simulink model "My_gfm_battery_sil_2_ConvIGBT_zDomain"  (R2025b)
settings: Solver=ode23t  StartTime=0.0  StopTime=10  MaxStep=1e-4  RelTol=1e-3
PreLoadFcn:
  | close all;
  | clear all;
  | clc;
  | 
  | 
  | modelDir = fileparts(get_param(bdroot,'FileName'));
  | 
  | load_system(fullfile(modelDir,'controls_element_lib.slx'));
  | load_system(fullfile(modelDir,'test_sequence_lib.slx'));
  | 
  | Simulink.importExternalCTypes('.\circuitControls_A_autogen.h')
InitFcn:
  | % frequency nominals
  | F_NOM = 60;
  | W_NOM = 2 * pi * F_NOM;
  | 
  | % base values relative to inverter
  | % --------------------------------
  | VLL_INV_NOM = 480;
  | P_INV_NOM = 1e6;
  | Q_INV_NOM = 0.5e6;
  | S_INV_NOM = sqrt(P_INV_NOM^2 + Q_INV_NOM^2);
  | 
  | I_INV_BASE = S_INV_NOM/(sqrt(3)*VLL_INV_NOM);
  | Z_INV_BASE = VLL_INV_NOM^2/S_INV_NOM;
  | L_INV_BASE = Z_INV_BASE / W_NOM;
  | C_INV_BASE = 1 / (Z_INV_BASE * W_NOM);
  | 
  | % nominal ratings for power system model
  | % --------------------------------------
  | INVERTER_COUNT = 100;
  | 
  | VLV_NOM = VLL_INV_NOM;
  | VMV_NOM = 35e3;
  | VHV_NOM = 230e3;
  | S_PLANT = INVERTER_COUNT * S_INV_NOM;
  | 
  | N_GSU = VHV_NOM/VMV_NOM;
  | N_MVT = VMV_NOM/VLV_NOM;
  | 
  | I_LV_BASE = S_PLANT/(sqrt(3)*VLV_NOM);
  | I_MV_BASE = S_PLANT/(sqrt(3)*VMV_NOM);
  | I_HV_BASE = S_PLANT/(sqrt(3)*VHV_NOM);
  | 
  | Z_LV_BASE = VLV_NOM^2/S_PLANT;
  | Z_MV_BASE = VMV_NOM^2/S_PLANT;
  | Z_HV_BASE = VHV_NOM^2/S_PLANT;
  | 
  | L_LV_BASE = Z_LV_BASE / W_NOM;
  | L_MV_BASE = Z_MV_BASE / W_NOM;
  | L_HV_BASE = Z_HV_BASE / W_NOM;
  | C_LV_BASE = 1 / (Z_LV_BASE * W_NOM);
  | C_MV_BASE = 1 / (Z_MV_BASE * W_NOM);
  | C_HV_BASE = 1 / (Z_HV_BASE * W_NOM);
undefined symbols (not defined in the file): D1, D11, Delta, gcbh, j, powergui, SampleTime, sps_rtmsupport, Ts
libraries: simulink x43, spsVoltageMeasurementLib x21, spsThreePhaseSeriesRLCBranchLib x20, spsControlledCurrentSourceLib x20, spsControlledVoltageSourceLib x15, spsThreePhaseVIMeasurementLib x12, spsSeriesRLCBranchLib x11, spsGroundLib x11, test_sequence_lib x10, controls_element_lib x9, spsCurrentMeasurementLib x8, spsThreePhaseTransformerTwoWindingsLib x6
(part 8 of 8)

== system My_gfm_battery_sil_2_ConvIGBT_zDomain/ac Network with MVT (native math)4/Two-Level Converter1/Model3 ==
  note: (Uref)
  g : Inport  SampleTime=Ts
  Block : Inport  Port=2
  Add : Sum  Inputs=+-
  Constant : Constant
  Constant1 : Constant  Value=0
  Constant2 : Constant
  Data Type Conversion2 : DataTypeConversion  OutDataTypeStr=double  SaturateOnIntegerOverflow=off  RndMeth=Floor
  Demux : Demux  Outputs=2
  Fcn2 : Fcn  Expr=(u(1)+1)*0.5
  MATLAB Function : MATLAB Function  TreatAsAtomicUnit=on
  Mux : Mux  Inputs=2
  Mux1 : Mux  Inputs=2
  Power : spsHalfBridgeModel/Power  SystemSampleTime=-1  VariantActivationTime=update diagram  EmptyChoice=off  PassThrough=off  PassThroughVariantControl=(default)  EmptyChoiceVariantControl=(default)  AllowFlexibleInterface=on  Latency=0  AutoFrameSizeCalculation=off
  Product2 : Product
  Product8 : Product
  Saturation : Saturate  UpperLimit=1.0  LowerLimit=-1.0
  Scope : Scope  NumInputPorts=2
      settings: ActiveDisplayYMinimum=-0.125  ActiveDisplayYMaximum=1.125
  Scope1 : Scope  NumInputPorts=2
      settings: ActiveDisplayYMinimum=-0.0256  ActiveDisplayYMaximum=0.96024  DataLoggingVariableName=ScopeData2
  Scope2 : Scope  NumInputPorts=5
      settings: ActiveDisplayYMinimum=-1250  ActiveDisplayYMaximum=1079.00943  DataLoggingVariableName=ScopeData3
  Switch : Switch  Criteria=u2 > Threshold  SaturateOnIntegerOverflow=off  InputSameDT=off
  Transfer Fcn : TransferFcn  Denominator=[1e-6 1]
  Transfer Fcn1 : TransferFcn  Denominator=[1e-6 1]
  Transfer Fcn2 : TransferFcn  Denominator=[1e-6 1]
  Voltage Measurement : spsVoltageMeasurementLib/Voltage Measurement  PhasorSimulation=off  OutputType=Complex  PSBequivalent=0
  + : PMIOPort  Tag=PMCPort  Side=Right
  - : PMIOPort  Tag=PMCPort  Port=2  Side=Right
  Out : PMIOPort  Tag=PMCPort  Port=3  Side=Left
  wires:
  Saturation/1 -> Fcn2/1
  g/1 -> Saturation/1
  Block/1 -> Switch/2, Scope/1
  Data Type Conversion2/1 -> Scope/2, Product2/1, Product8/1
  Product2/1 -> Mux1/1
  Product8/1 -> Mux1/2
  Add/1 -> Scope1/2, Product8/2
  Constant/1 -> Add/1
  Fcn2/1 -> Add/2, Scope1/1, Product2/2
  Switch/1 -> Data Type Conversion2/1
  Power/2 -> Scope2/4, Demux/1
  Demux/2 -> Transfer Fcn2/1
  Demux/1 -> Transfer Fcn/1
  Transfer Fcn/1 -> Mux/1
  Transfer Fcn2/1 -> Mux/2
  Mux/1 -> MATLAB Function/3(I)
  Transfer Fcn1/1 -> MATLAB Function/2(Vdc)
  Power/1 -> Scope2/2, Transfer Fcn1/1
  MATLAB Function/2(Idc) -> Power/2, Scope2/3
  MATLAB Function/1(V) -> Power/1, Scope2/1
  Mux1/1 -> MATLAB Function/1(g)
  Constant1/1 -> Switch/1
  Constant2/1 -> Switch/3
  Voltage Measurement/1 -> Scope2/5
  connections:
  Out/RConn1 -- Power/LConn1 -- Voltage Measurement/LConn1
  -/RConn1 -- Power/RConn2 -- Voltage Measurement/LConn2
  Power/RConn1 -- +/RConn1

== system My_gfm_battery_sil_2_ConvIGBT_zDomain/ac Network with MVT (native math)4/powergui/EquivalentModel1 ==
  Sources : Subsystem
  State-Space : S-Function  FunctionName=sfun_spid_contc  Parameters=S.Mg, [S.nb.x S.nb.u S.nb.y S.nb.s], S.x0, S.MgColNames  SFunctionDeploymentMode=off  EnableBusSupport=off
  Yout : Subsystem
  wires:
  State-Space/1 -> Yout/1(v,i)
  Sources/1(u) -> State-Space/1

== system My_gfm_battery_sil_2_ConvIGBT_zDomain/ac Network with MVT (native math)4/powergui/EquivalentModel2 ==
  Sources : Subsystem
  State-Space : S-Function  FunctionName=sfun_spid_contc  Parameters=S.Mg, [S.nb.x S.nb.u S.nb.y S.nb.s], S.x0, S.MgColNames  SFunctionDeploymentMode=off  EnableBusSupport=off
  Yout : Subsystem
  wires:
  State-Space/1 -> Yout/1(v,i)
  Sources/1(u) -> State-Space/1

== system My_gfm_battery_sil_2_ConvIGBT_zDomain/ac Network with MVT (native math)4/powergui/EquivalentModel3 ==
  Sources : Subsystem
  State-Space : S-Function  FunctionName=sfun_spid_contc  Parameters=S.Mg, [S.nb.x S.nb.u S.nb.y S.nb.s], S.x0, S.MgColNames  SFunctionDeploymentMode=off  EnableBusSupport=off
  Yout : Subsystem
  wires:
  State-Space/1 -> Yout/1(v,i)
  Sources/1(u) -> State-Space/1

== system My_gfm_battery_sil_2_ConvIGBT_zDomain/ac Network with MVT (native math)5/filter_caps/LPF1 ==
  in : Inport
  rst : Inport  Port=2
  Constant : Constant  Value=0
  Constant2 : Constant  Value=Ts
  Delay : Delay  DelayLength=1  InitialCondition=0
  Logical Operator : Logic  Operator=NOT  AllPortsSameDT=off  OutDataTypeStr=boolean
  Product : Product
  Sum : Sum  Inputs=|++
  Switch : Switch  Criteria=u2 ~= 0  SaturateOnIntegerOverflow=off  InputSameDT=off
  out : Outport
  FB : Outport  Port=2
  wires:
  Delay/1 -> Sum/2, FB/1
  Switch/1 -> out/1, Delay/1
  in/1 -> Product/2
  Product/1 -> Sum/1
  Constant2/1 -> Product/1
  Sum/1 -> Switch/1
  Constant/1 -> Switch/3
  rst/1 -> Logical Operator/1
  Logical Operator/1 -> Switch/2

== system My_gfm_battery_sil_2_ConvIGBT_zDomain/ac Network with MVT (native math)5/filter_inductors/LPF1 ==
  in : Inport
  rst : Inport  Port=2
  Constant : Constant  Value=0
  Constant2 : Constant  Value=Ts
  Delay : Delay  DelayLength=1  InitialCondition=0
  Logical Operator : Logic  Operator=NOT  AllPortsSameDT=off  OutDataTypeStr=boolean
  Product : Product
  Sum : Sum  Inputs=|++
  Switch : Switch  Criteria=u2 ~= 0  SaturateOnIntegerOverflow=off  InputSameDT=off
  out : Outport
  FB : Outport  Port=2
  wires:
  Delay/1 -> Sum/2, FB/1
  Switch/1 -> out/1, Delay/1
  in/1 -> Product/2
  Product/1 -> Sum/1
  Constant2/1 -> Product/1
  Sum/1 -> Switch/1
  Constant/1 -> Switch/3
  rst/1 -> Logical Operator/1
  Logical Operator/1 -> Switch/2

== system My_gfm_battery_sil_2_ConvIGBT_zDomain/ac Network with MVT (native math)5/solver_LPF2/LPF1 ==
  in : Inport
  rst : Inport  Port=2
  Constant : Constant  Value=0
  Constant2 : Constant  Value=Ts
  Delay : Delay  DelayLength=1  InitialCondition=0
  Logical Operator : Logic  Operator=NOT  AllPortsSameDT=off  OutDataTypeStr=boolean
  Product : Product
  Sum : Sum  Inputs=|++
  Switch : Switch  Criteria=u2 ~= 0  SaturateOnIntegerOverflow=off  InputSameDT=off
  out : Outport
  FB : Outport  Port=2
  wires:
  Delay/1 -> Sum/2, FB/1
  Switch/1 -> out/1, Delay/1
  in/1 -> Product/2
  Product/1 -> Sum/1
  Constant2/1 -> Product/1
  Sum/1 -> Switch/1
  Constant/1 -> Switch/3
  rst/1 -> Logical Operator/1
  Logical Operator/1 -> Switch/2

== system My_gfm_battery_sil_2_ConvIGBT_zDomain/ac Network with MVT (native math)5/solver_LPF4/LPF1 ==
  in : Inport
  rst : Inport  Port=2
  Constant : Constant  Value=0
  Constant2 : Constant  Value=Ts
  Delay : Delay  DelayLength=1  InitialCondition=0
  Logical Operator : Logic  Operator=NOT  AllPortsSameDT=off  OutDataTypeStr=boolean
  Product : Product
  Sum : Sum  Inputs=|++
  Switch : Switch  Criteria=u2 ~= 0  SaturateOnIntegerOverflow=off  InputSameDT=off
  out : Outport
  FB : Outport  Port=2
  wires:
  Delay/1 -> Sum/2, FB/1
  Switch/1 -> out/1, Delay/1
  in/1 -> Product/2
  Product/1 -> Sum/1
  Constant2/1 -> Product/1
  Sum/1 -> Switch/1
  Constant/1 -> Switch/3
  rst/1 -> Logical Operator/1
  Logical Operator/1 -> Switch/2

== system My_gfm_battery_sil_2_ConvIGBT_zDomain/My Inverter Controller /My_acMonitor_A/Analyzer_V/complex_LPF ==
  note: This was needed because Simulink complains when using transfer functions directly on arrays or complex numbers.
  In1 : Inport
  Complex to Real-Imag : ComplexToRealImag
  Gain2 : Gain  Gain=1/tau
  Gain3 : Gain  Gain=1/tau
  Integrator : Integrator
  Integrator1 : Integrator
  Real-Imag to Complex : RealImagToComplex
  Sum : Sum  Inputs=|+-
  Sum1 : Sum  Inputs=|+-
  Out1 : Outport
  wires:
  Real-Imag to Complex/1 -> Out1/1
  In1/1 -> Complex to Real-Imag/1
  Complex to Real-Imag/1 -> Sum/1
  Integrator/1 -> Real-Imag to Complex/1, Sum/2
  Sum1/1 -> Gain3/1
  Complex to Real-Imag/2 -> Sum1/1
  Gain2/1 -> Integrator/1
  Sum/1 -> Gain2/1
  Integrator1/1 -> Sum1/2, Real-Imag to Complex/2
  Gain3/1 -> Integrator1/1

== system My_gfm_battery_sil_2_ConvIGBT_zDomain/My Inverter Controller /My_acMonitor_A/Analyzer_V1/complex_LPF ==
  note: This was needed because Simulink complains when using transfer functions directly on arrays or complex numbers.
  In1 : Inport
  Complex to Real-Imag : ComplexToRealImag
  Gain2 : Gain  Gain=1/tau
  Gain3 : Gain  Gain=1/tau
  Integrator : Integrator
  Integrator1 : Integrator
  Real-Imag to Complex : RealImagToComplex
  Sum : Sum  Inputs=|+-
  Sum1 : Sum  Inputs=|+-
  Out1 : Outport
  wires:
  Real-Imag to Complex/1 -> Out1/1
  In1/1 -> Complex to Real-Imag/1
  Complex to Real-Imag/1 -> Sum/1
  Integrator/1 -> Real-Imag to Complex/1, Sum/2
  Sum1/1 -> Gain3/1
  Complex to Real-Imag/2 -> Sum1/1
  Gain2/1 -> Integrator/1
  Sum/1 -> Gain2/1
  Integrator1/1 -> Sum1/2, Real-Imag to Complex/2
  Gain3/1 -> Integrator1/1

== system My_gfm_battery_sil_2_ConvIGBT_zDomain/My Inverter Controller /My_acMonitor_A/PLL_3ph/oscillator_3ph ==
  f : Inport
  Cos : Trigonometry  Operator=cos
  Gain : Gain  Gain=2*pi
  Integrator : Integrator
  Real-Imag to Complex : RealImagToComplex
  Sin : Trigonometry
  Sum1 : Sum  Inputs=|++
  phase_shift : Constant  Value=[0 -1/3 -2/3]
  osc[3] : Outport
  wires:
  Sum1/1 -> Gain/1
  phase_shift/1 -> Sum1/2
  Sin/1 -> Real-Imag to Complex/2
  Integrator/1 -> Sum1/1
  Gain/1 -> Sin/1, Cos/1
  Cos/1 -> Real-Imag to Complex/1
  Real-Imag to Complex/1 -> osc[3]/1
  f/1 -> Integrator/1

== system My_gfm_battery_sil_2_ConvIGBT_zDomain/My Inverter Controller /My_circuit_controls_A2/SOGI/Integrator1 ==
  In : Inport
  Ts : Inport  Port=2
  Delay1 : Delay  DelayLength=1
  Delay2 : Delay  DelayLength=1
  Delay3 : Delay  DelayLength=1
  Gain : Gain  Gain=1/12
  Gain1 : Gain  Gain=23
  Gain2 : Gain  Gain=16
  Gain3 : Gain  Gain=5
  Product : Product
  Sum : Sum  Inputs=|+-
  Sum1 : Sum  Inputs=|++
  Sum2 : Sum  Inputs=|++
  Out : Outport  VectorParamsAs1DForOutWhenUnconnected=off
  wires:
  Delay2/1 -> Gain2/1, Delay3/1
  Delay1/1 -> Sum2/2, Gain1/1, Delay2/1
  Delay3/1 -> Gain3/1
  Gain2/1 -> Sum/2
  Gain1/1 -> Sum/1
  Gain3/1 -> Sum1/2
  Sum/1 -> Sum1/1
  Gain/1 -> Sum2/1
  Sum2/1 -> Delay1/1
  Product/1 -> Gain/1
  Sum1/1 -> Out/1
  Ts/1 -> Product/2
  In/1 -> Product/1

== system My_gfm_battery_sil_2_ConvIGBT_zDomain/My Inverter Controller /My_circuit_controls_A2/SOGI/Integrator3 ==
  In : Inport
  Ts : Inport  Port=2
  Delay1 : Delay  DelayLength=1
  Delay2 : Delay  DelayLength=1
  Delay3 : Delay  DelayLength=1
  Gain : Gain  Gain=1/12
  Gain1 : Gain  Gain=23
  Gain2 : Gain  Gain=16
  Gain3 : Gain  Gain=5
  Product : Product
  Sum : Sum  Inputs=|+-
  Sum1 : Sum  Inputs=|++
  Sum2 : Sum  Inputs=|++
  Out : Outport  VectorParamsAs1DForOutWhenUnconnected=off
  wires:
  Delay2/1 -> Gain2/1, Delay3/1
  Delay1/1 -> Sum2/2, Gain1/1, Delay2/1
  Delay3/1 -> Gain3/1
  Gain2/1 -> Sum/2
  Gain1/1 -> Sum/1
  Gain3/1 -> Sum1/2
  Sum/1 -> Sum1/1
  Gain/1 -> Sum2/1
  Sum2/1 -> Delay1/1
  Product/1 -> Gain/1
  Sum1/1 -> Out/1
  Ts/1 -> Product/2
  In/1 -> Product/1

== system My_gfm_battery_sil_2_ConvIGBT_zDomain/My Inverter Controller /My_circuit_controls_A2/Subsystem/LPF4 ==
  note: Forward integrator
  in : Inport
  Constant2 : Constant  Value=Ts
  Constant3 : Constant  Value=OmegaUp
  Constant4 : Constant  Value=OmegaDn
  Constant9 : Constant  Value=1/20000
  Delay : Delay  DelayLength=1  InitialCondition=0
  Gain : Gain  Gain=1/5
  Math Function : Math  Operator=reciprocal  SignedPower=on
  MinMax : MinMax  Function=max  Inputs=2
  MinMax1 : MinMax  Inputs=2
  MinMax2 : MinMax  Inputs=2
  Product : Product
  Product1 : Product
  Product2 : Product
  Saturation : Saturate  UpperLimit=inf  LowerLimit=0
  Saturation1 : Saturate  UpperLimit=0  LowerLimit=-inf
  Sum : Sum  Inputs=|++
  Sum1 : Sum  Inputs=|++
  Sum4 : Sum  Inputs=|+-
  out : Outport
  wires:
  Delay/1 -> Sum4/2, Sum/2
  in/1 -> Sum4/1
  Sum4/1 -> Product2/1, Product1/2
  Sum/1 -> out/1, Delay/1
  Saturation/1 -> Sum1/1
  Saturation1/1 -> Sum1/2
  Sum1/1 -> Product/2
  Product/1 -> Sum/1
  [Ts] -> Product/1
  [OmegaUp] -> Product1/1
  [OmegaDn] -> Product2/2
  Constant2/1 -> MinMax/1
  MinMax/1 -> [Ts]
  Constant9/1 -> MinMax/2
  MinMax1/1 -> [OmegaUp]
  MinMax2/1 -> [OmegaDn]
  [Ts] -> Math Function/1
  Math Function/1 -> Gain/1
  Gain/1 -> MinMax1/2, MinMax2/1
  Constant3/1 -> MinMax1/1
  Constant4/1 -> MinMax2/2
  Product1/1 -> Saturation/1
  Product2/1 -> Saturation1/1

== system My_gfm_battery_sil_2_ConvIGBT_zDomain/My Inverter Controller /My_circuit_controls_A2/virtual damper/Damping HPF ==
  note: Forward integrator
  in : Inport
  Constant2 : Constant  Value=Ts
  Constant3 : Constant  Value=OmegaUp
  Constant4 : Constant  Value=OmegaDn
  Constant9 : Constant  Value=1/20000
  Delay : Delay  DelayLength=1  InitialCondition=0
  Gain : Gain  Gain=1/5
  Math Function : Math  Operator=reciprocal  SignedPower=on
  MinMax : MinMax  Function=max  Inputs=2
  MinMax1 : MinMax  Inputs=2
  MinMax2 : MinMax  Inputs=2
  Product : Product
  Product1 : Product
  Product2 : Product
  Saturation : Saturate  UpperLimit=inf  LowerLimit=0
  Saturation1 : Saturate  UpperLimit=0  LowerLimit=-inf
  Sum : Sum  Inputs=|+-
  Sum1 : Sum  Inputs=|++
  Sum2 : Sum  Inputs=|++
  Sum3 : Sum  Inputs=|+-
  out : Outport  VectorParamsAs1DForOutWhenUnconnected=off
  wires:
  Gain/1 -> MinMax1/2, MinMax2/1
  [Ts] -> Product/1
  [Ts] -> Math Function/1
  Delay/1 -> Sum1/2, Sum/2
  MinMax1/1 -> [OmegaUp]
  Constant9/1 -> MinMax/2
  Sum/1 -> Product2/1, Product1/2
  Math Function/1 -> Gain/1
  Constant4/1 -> MinMax2/2
  Constant2/1 -> MinMax/1
  Saturation/1 -> Sum2/1
  Sum1/1 -> Sum3/2, Delay/1
  Sum2/1 -> Product/2
  MinMax2/1 -> [OmegaDn]
  Product/1 -> Sum1/1
  [OmegaUp] -> Product1/1
  Constant3/1 -> MinMax1/1
  MinMax/1 -> [Ts]
  Product2/1 -> Saturation1/1
  in/1 -> Sum3/1, Sum/1
  Product1/1 -> Saturation/1
  [OmegaDn] -> Product2/2
  Saturation1/1 -> Sum2/2
  Sum3/1 -> out/1

== system My_gfm_battery_sil_2_ConvIGBT_zDomain/My Inverter Controller /My_circuit_controls_A4/SOGI/Integrator1 ==
  In : Inport
  Ts : Inport  Port=2
  Delay1 : Delay  DelayLength=1
  Delay2 : Delay  DelayLength=1
  Delay3 : Delay  DelayLength=1
  Gain : Gain  Gain=1/12
  Gain1 : Gain  Gain=23
  Gain2 : Gain  Gain=16
  Gain3 : Gain  Gain=5
  Product : Product
  Sum : Sum  Inputs=|+-
  Sum1 : Sum  Inputs=|++
  Sum2 : Sum  Inputs=|++
  Out : Outport  VectorParamsAs1DForOutWhenUnconnected=off
  wires:
  Delay2/1 -> Gain2/1, Delay3/1
  Delay1/1 -> Sum2/2, Gain1/1, Delay2/1
  Delay3/1 -> Gain3/1
  Gain2/1 -> Sum/2
  Gain1/1 -> Sum/1
  Gain3/1 -> Sum1/2
  Sum/1 -> Sum1/1
  Gain/1 -> Sum2/1
  Sum2/1 -> Delay1/1
  Product/1 -> Gain/1
  Sum1/1 -> Out/1
  Ts/1 -> Product/2
  In/1 -> Product/1

== system My_gfm_battery_sil_2_ConvIGBT_zDomain/My Inverter Controller /My_circuit_controls_A4/SOGI/Integrator3 ==
  In : Inport
  Ts : Inport  Port=2
  Delay1 : Delay  DelayLength=1
  Delay2 : Delay  DelayLength=1
  Delay3 : Delay  DelayLength=1
  Gain : Gain  Gain=1/12
  Gain1 : Gain  Gain=23
  Gain2 : Gain  Gain=16
  Gain3 : Gain  Gain=5
  Product : Product
  Sum : Sum  Inputs=|+-
  Sum1 : Sum  Inputs=|++
  Sum2 : Sum  Inputs=|++
  Out : Outport  VectorParamsAs1DForOutWhenUnconnected=off
  wires:
  Delay2/1 -> Gain2/1, Delay3/1
  Delay1/1 -> Sum2/2, Gain1/1, Delay2/1
  Delay3/1 -> Gain3/1
  Gain2/1 -> Sum/2
  Gain1/1 -> Sum/1
  Gain3/1 -> Sum1/2
  Sum/1 -> Sum1/1
  Gain/1 -> Sum2/1
  Sum2/1 -> Delay1/1
  Product/1 -> Gain/1
  Sum1/1 -> Out/1
  Ts/1 -> Product/2
  In/1 -> Product/1

== system My_gfm_battery_sil_2_ConvIGBT_zDomain/My Inverter Controller /My_circuit_controls_A4/Subsystem/LPF4 ==
  note: Forward integrator
  in : Inport
  Constant2 : Constant  Value=Ts
  Constant3 : Constant  Value=OmegaUp
  Constant4 : Constant  Value=OmegaDn
  Constant9 : Constant  Value=1/20000
  Delay : Delay  DelayLength=1  InitialCondition=0
  Gain : Gain  Gain=1/5
  Math Function : Math  Operator=reciprocal  SignedPower=on
  MinMax : MinMax  Function=max  Inputs=2
  MinMax1 : MinMax  Inputs=2
  MinMax2 : MinMax  Inputs=2
  Product : Product
  Product1 : Product
  Product2 : Product
  Saturation : Saturate  UpperLimit=inf  LowerLimit=0
  Saturation1 : Saturate  UpperLimit=0  LowerLimit=-inf
  Sum : Sum  Inputs=|++
  Sum1 : Sum  Inputs=|++
  Sum4 : Sum  Inputs=|+-
  out : Outport
  wires:
  Delay/1 -> Sum4/2, Sum/2
  in/1 -> Sum4/1
  Sum4/1 -> Product2/1, Product1/2
  Sum/1 -> out/1, Delay/1
  Saturation/1 -> Sum1/1
  Saturation1/1 -> Sum1/2
  Sum1/1 -> Product/2
  Product/1 -> Sum/1
  [Ts] -> Product/1
  [OmegaUp] -> Product1/1
  [OmegaDn] -> Product2/2
  Constant2/1 -> MinMax/1
  MinMax/1 -> [Ts]
  Constant9/1 -> MinMax/2
  MinMax1/1 -> [OmegaUp]
  MinMax2/1 -> [OmegaDn]
  [Ts] -> Math Function/1
  Math Function/1 -> Gain/1
  Gain/1 -> MinMax1/2, MinMax2/1
  Constant3/1 -> MinMax1/1
  Constant4/1 -> MinMax2/2
  Product1/1 -> Saturation/1
  Product2/1 -> Saturation1/1

== system My_gfm_battery_sil_2_ConvIGBT_zDomain/My Inverter Controller /My_circuit_controls_A4/virtual damper/Damping HPF ==
  note: Forward integrator
  in : Inport
  Constant2 : Constant  Value=Ts
  Constant3 : Constant  Value=OmegaUp
  Constant4 : Constant  Value=OmegaDn
  Constant9 : Constant  Value=1/20000
  Delay : Delay  DelayLength=1  InitialCondition=0
  Gain : Gain  Gain=1/5
  Math Function : Math  Operator=reciprocal  SignedPower=on
  MinMax : MinMax  Function=max  Inputs=2
  MinMax1 : MinMax  Inputs=2
  MinMax2 : MinMax  Inputs=2
  Product : Product
  Product1 : Product
  Product2 : Product
  Saturation : Saturate  UpperLimit=inf  LowerLimit=0
  Saturation1 : Saturate  UpperLimit=0  LowerLimit=-inf
  Sum : Sum  Inputs=|+-
  Sum1 : Sum  Inputs=|++
  Sum2 : Sum  Inputs=|++
  Sum3 : Sum  Inputs=|+-
  out : Outport  VectorParamsAs1DForOutWhenUnconnected=off
  wires:
  Gain/1 -> MinMax1/2, MinMax2/1
  [Ts] -> Product/1
  [Ts] -> Math Function/1
  Delay/1 -> Sum1/2, Sum/2
  MinMax1/1 -> [OmegaUp]
  Constant9/1 -> MinMax/2
  Sum/1 -> Product2/1, Product1/2
  Math Function/1 -> Gain/1
  Constant4/1 -> MinMax2/2
  Constant2/1 -> MinMax/1
  Saturation/1 -> Sum2/1
  Sum1/1 -> Sum3/2, Delay/1
  Sum2/1 -> Product/2
  MinMax2/1 -> [OmegaDn]
  Product/1 -> Sum1/1
  [OmegaUp] -> Product1/1
  Constant3/1 -> MinMax1/1
  MinMax/1 -> [Ts]
  Product2/1 -> Saturation1/1
  in/1 -> Sum3/1, Sum/1
  Product1/1 -> Saturation/1
  [OmegaDn] -> Product2/2
  Saturation1/1 -> Sum2/2
  Sum3/1 -> out/1

== system My_gfm_battery_sil_2_ConvIGBT_zDomain/My Inverter Controller /My_currentLimiting_B/Current_foldback1/LPF  ==
  In : Inport
  1/0.01 : Gain  Gain=1/0.01
  Integrator : Integrator
  Sum3 : Sum  Inputs=|+-
  Out : Outport
  wires:
  Integrator/1 -> Out/1, Sum3/2
  Sum3/1 -> 1/0.01/1
  In/1 -> Sum3/1
  1/0.01/1 -> Integrator/1

== system My_gfm_battery_sil_2_ConvIGBT_zDomain/My Inverter Controller /My_machineModel_A/AVR/ Saturation ==
  In : Inport
  Complex to Real-Imag : ComplexToRealImag
  Real-Imag to Complex3 : RealImagToComplex
  Saturation3 : Saturate  UpperLimit=0.1*VllRated  LowerLimit=-0.1*VllRated
  Saturation4 : Saturate  UpperLimit=0.1*VllRated  LowerLimit=-0.1*VllRated
  Out : Outport  VectorParamsAs1DForOutWhenUnconnected=off
  wires:
  Complex to Real-Imag/1 -> Saturation3/1
  Saturation4/1 -> Real-Imag to Complex3/2
  Complex to Real-Imag/2 -> Saturation4/1
  Saturation3/1 -> Real-Imag to Complex3/1
  In/1 -> Complex to Real-Imag/1
  Real-Imag to Complex3/1 -> Out/1

== system My_gfm_battery_sil_2_ConvIGBT_zDomain/My Inverter Controller /My_machineModel_A/AVR/LPF ==
  In : Inport
  1/tauMeas : Gain  Gain=1/tauMeas
  Integrator : Integrator
  Sum3 : Sum  Inputs=|+-
  Out : Outport
  wires:
  Integrator/1 -> Out/1, Sum3/2
  Sum3/1 -> 1/tauMeas/1
  In/1 -> Sum3/1
  1/tauMeas/1 -> Integrator/1

== system My_gfm_battery_sil_2_ConvIGBT_zDomain/My Inverter Controller /My_machineModel_A/AVR/LPF  ==
  In : Inport
  1/tauMeas : Gain  Gain=1/tauMeas
  Integrator : Integrator
  Sum3 : Sum  Inputs=|+-
  Out : Outport
  wires:
  Integrator/1 -> Out/1, Sum3/2
  Sum3/1 -> 1/tauMeas/1
  In/1 -> Sum3/1
  1/tauMeas/1 -> Integrator/1

== system My_gfm_battery_sil_2_ConvIGBT_zDomain/My Inverter Controller /My_machineModel_A/AVR/LPF   ==
  In : Inport
  1/tauMeas : Gain  Gain=1/tauMeas
  Integrator : Integrator
  Sum3 : Sum  Inputs=|+-
  Out : Outport
  wires:
  Integrator/1 -> Out/1, Sum3/2
  Sum3/1 -> 1/tauMeas/1
  In/1 -> Sum3/1
  1/tauMeas/1 -> Integrator/1

== system My_gfm_battery_sil_2_ConvIGBT_zDomain/My Inverter Controller /My_machineModel_A/AVR/assymmetric filter ==
  note: The saturation block is configured to cause a rapid rise, but much slow drop in output.
  in : Inport
  Gain1 : Gain  Gain=1/tauBkSt
  Integrator : Integrator
  Saturation1 : Saturate  UpperLimit=VllRated  LowerLimit=-0.02 * VllRated
  Sum3 : Sum  Inputs=|+-
  out : Outport
  wires:
  Saturation1/1 -> Integrator/1
  Gain1/1 -> Saturation1/1
  in/1 -> Sum3/1
  Sum3/1 -> Gain1/1
  Integrator/1 -> Sum3/2, out/1

== system My_gfm_battery_sil_2_ConvIGBT_zDomain/My Inverter Controller /My_machineModel_A/AVR/current analyzer ==
  osc[3] : Inport
  iac : Inport  Port=2
  Complex to Real-Imag : ComplexToRealImag
  Conj : Math  Operator=conj  SignedPower=on
  Product1 : Product
  Product2 : Product
  Sum of Elements1 : Sum  Inputs=+
  Sum of Elements2 : Sum  Inputs=+
  Transfer Fcn : TransferFcn  Denominator=[0.02 1]
  Transfer Fcn1 : TransferFcn  Denominator=[0.02 1]
  over_sqrt(3) : Gain  Gain=1/sqrt(3)
  over_sqrt(3)1 : Gain  Gain=1/sqrt(3)
  sqrt(2) : Gain  Gain=sqrt(2)
  Id : Outport
  Iq : Outport  Port=2
  wires:
  Transfer Fcn/1 -> Iq/1
  osc[3]/1 -> Conj/1
  Transfer Fcn1/1 -> Id/1
  over_sqrt(3)1/1 -> Transfer Fcn1/1
  over_sqrt(3)/1 -> Transfer Fcn/1
  Complex to Real-Imag/1 -> Product2/1
  Complex to Real-Imag/2 -> Product1/1
  Sum of Elements2/1 -> over_sqrt(3)1/1
  iac/1 -> Product2/2, Product1/2
  Product1/1 -> Sum of Elements1/1
  Sum of Elements1/1 -> over_sqrt(3)/1
  sqrt(2)/1 -> Complex to Real-Imag/1
  Conj/1 -> sqrt(2)/1
  Product2/1 -> Sum of Elements2/1

== system My_gfm_battery_sil_2_ConvIGBT_zDomain/My Inverter Controller /My_machineModel_A/Exciter/LPF ==
  In : Inport
  Integrator : Integrator
  Sum3 : Sum  Inputs=|+-
  wExciter : Gain  Gain=wExciter
  Out : Outport
  wires:
  Integrator/1 -> Out/1, Sum3/2
  Sum3/1 -> wExciter/1
  In/1 -> Sum3/1
  wExciter/1 -> Integrator/1

== system My_gfm_battery_sil_2_ConvIGBT_zDomain/My Inverter Controller /My_machineModel_A/Exciter/modulator ==
  cmd : Inport
  osc : Inport  Port=2
  Complex to Real-Imag : ComplexToRealImag
  Complex to Real-Imag1 : ComplexToRealImag
  Gain : Gain  Gain=sqrt(2)
  Product1 : Product
  Product2 : Product
  Sum1 : Sum  Inputs=|+-
  ref : Outport
  wires:
  osc/1 -> Gain/1
  Complex to Real-Imag/1 -> Product2/2
  Product2/1 -> Sum1/1
  Sum1/1 -> ref/1  "i"
  Gain/1 -> Complex to Real-Imag/1
  Complex to Real-Imag/2 -> Product1/2
  Product1/1 -> Sum1/2
  cmd/1 -> Complex to Real-Imag1/1
  Complex to Real-Imag1/1 -> Product2/1
  Complex to Real-Imag1/2 -> Product1/1

== system My_gfm_battery_sil_2_ConvIGBT_zDomain/My Inverter Controller /My_machineModel_A/governer/LPF(DamperDecoupler) limited  ==
  In : Inport
  Constant : Constant  Value=1/tau_damp
  Constant1 : Constant  Value=wGoverner
  Integrator : Integrator  LimitOutput=on  UpperSaturationLimit=1.2*SRated  LowerSaturationLimit=-1.2*SRated
  MinMax : MinMax  Inputs=2
  Product : Product
  Sum3 : Sum  Inputs=|+-
  Out : Outport
  wires:
  Integrator/1 -> Out/1, Sum3/2
  Sum3/1 -> Product/2
  In/1 -> Sum3/1
  Product/1 -> Integrator/1
  MinMax/1 -> Product/1
  Constant/1 -> MinMax/1
  Constant1/1 -> MinMax/2

== system My_gfm_battery_sil_2_ConvIGBT_zDomain/My Inverter Controller /My_machineModel_A/governer/synchronizer ==
  note: Big Range?
  note: prevent it from acting during typical faults
  note: Prevent loss of sync at low voltage events, using asym filter to traget long extended low voltage events
  note: Keeps the machine spining in synchronize while machine is disabled, disabling the machine means
  note: Why?
  Vq : Inport
  Vt : Inport  Port=2
  machine_enabled : Inport  Port=3
  Constant : Constant
  Gain : Gain  Gain=SRated
  Gain2 : Gain  Gain=1/VllRated
  "HPF " : Subsystem
  Product1 : Product
  Saturation : Saturate  UpperLimit=1  LowerLimit=0
  Sum : Sum  Inputs=|++
  Sum2 : Sum  Inputs=|+-
  Switch : Switch  Criteria=u2 > Threshold  SaturateOnIntegerOverflow=off  InputSameDT=off
  assymmetric filter1 : Subsystem
  gain : Gain  Gain=wSync
  kFastSync : Gain  Gain=kpFastSync
  kSync : Gain  Gain=kpSync
  pSyncLimit : Saturate  UpperLimit=3  LowerLimit=-3
  syncFadeGain : Gain  Gain=kpSyncFade
  syncFadeThreshold : Constant  Value=SyncFadeThres
  to_pu : Gain  Gain=1 / VllRated
  p_sync_pu : Outport
  wires:
  to_pu/1 -> Sum2/2
  Vt/1 -> assymmetric filter1/1(in)
  assymmetric filter1/1(out) -> to_pu/1
  pSyncLimit/1 -> Gain/1
  kSync/1 -> Sum/1
  Sum/1 -> pSyncLimit/1
  Product1/1 -> p_sync_pu/1
  Constant/1 -> Switch/3
  Sum2/1 -> syncFadeGain/1
  machine_enabled/1 -> Switch/2
  syncFadeGain/1 -> Saturation/1
  Saturation/1 -> Switch/1
  syncFadeThreshold/1 -> Sum2/1
  Switch/1 -> Product1/2
  Gain2/1 -> kFastSync/1, kSync/1
  Vq/1 -> Gain2/1
  Gain/1 -> Product1/1  "p_sync"
  kFastSync/1 -> "HPF "/1(in)
  "HPF "/1(out) -> gain/1
  gain/1 -> Sum/2

== system My_gfm_battery_sil_2_ConvIGBT_zDomain/My Inverter Controller /My_machineModel_A/rotor model/HPF (wDamperDecoupler) 1 ==
  in : Inport
  1/tau_damp : Gain  Gain=1/tau_damp
  Integrator : Integrator
  Sum : Sum  Inputs=|+-
  out : Outport
  wires:
  Sum/1 -> out/1, 1/tau_damp/1
  in/1 -> Sum/1
  Integrator/1 -> Sum/2
  1/tau_damp/1 -> Integrator/1

== system My_gfm_battery_sil_2_ConvIGBT_zDomain/My Inverter Controller /My_machineModel_A/rotor model/oscillator_3ph ==
  f : Inport
  Cos : Trigonometry  Operator=cos
  Gain : Gain  Gain=2*pi
  Integrator : Integrator
  Real-Imag to Complex : RealImagToComplex
  Sin : Trigonometry
  Sum1 : Sum  Inputs=|++
  phase_shift : Constant  Value=[0 -1/3 -2/3]
  osc[3] : Outport
  wires:
  f/1 -> Integrator/1
  Real-Imag to Complex/1 -> osc[3]/1
  Cos/1 -> Real-Imag to Complex/1
  Gain/1 -> Cos/1, Sin/1
  Integrator/1 -> Sum1/1
  Sin/1 -> Real-Imag to Complex/2
  phase_shift/1 -> Sum1/2
  Sum1/1 -> Gain/1

== system My_gfm_battery_sil_2_ConvIGBT_zDomain/My Inverter Controller /My_machineModel_A/voltage analyzer/LPF ==
  In : Inport
  1/tauMeas : Gain  Gain=1/tauMeas
  Integrator : Integrator
  Sum3 : Sum  Inputs=|+-
  Out : Outport
  wires:
  Integrator/1 -> Out/1, Sum3/2
  Sum3/1 -> 1/tauMeas/1
  In/1 -> Sum3/1
  1/tauMeas/1 -> Integrator/1

== system My_gfm_battery_sil_2_ConvIGBT_zDomain/My Inverter Controller /My_machineModel_A/voltage analyzer/LPF  ==
  In : Inport
  1/tauMeas : Gain  Gain=1/tauMeas
  Integrator : Integrator
  Sum3 : Sum  Inputs=|+-
  Out : Outport
  wires:
  Integrator/1 -> Out/1, Sum3/2
  Sum3/1 -> 1/tauMeas/1
  In/1 -> Sum3/1
  1/tauMeas/1 -> Integrator/1

== system My_gfm_battery_sil_2_ConvIGBT_zDomain/My Inverter Controller /My_machineModel_A1/excitation/LPF ==
  In : Inport
  Integrator : Integrator
  Sum3 : Sum  Inputs=|+-
  wExciter : Gain  Gain=wExciter
  Out : Outport
  wires:
  Integrator/1 -> Out/1, Sum3/2
  Sum3/1 -> wExciter/1
  In/1 -> Sum3/1
  wExciter/1 -> Integrator/1

== system My_gfm_battery_sil_2_ConvIGBT_zDomain/My Inverter Controller /My_machineModel_A1/excitation/assymmetric filter1 ==
  note: The saturation block is configured to cause a rapid rise, but much slow drop in output.
  in : Inport
  Gain1 : Gain  Gain=2
  Integrator : Integrator
  Saturation1 : Saturate  UpperLimit=VllRated  LowerLimit=-0.02 * VllRated
  Sum3 : Sum  Inputs=|+-
  out : Outport
  wires:
  Saturation1/1 -> Integrator/1
  Gain1/1 -> Saturation1/1
  in/1 -> Sum3/1
  Sum3/1 -> Gain1/1
  Integrator/1 -> Sum3/2, out/1

== system My_gfm_battery_sil_2_ConvIGBT_zDomain/My Inverter Controller /My_machineModel_A1/excitation/modulator ==
  cmd : Inport
  osc : Inport  Port=2
  Complex to Real-Imag : ComplexToRealImag
  Complex to Real-Imag1 : ComplexToRealImag
  Gain : Gain  Gain=sqrt(2)
  Product1 : Product
  Product2 : Product
  Sum1 : Sum  Inputs=|+-
  ref : Outport
  wires:
  osc/1 -> Gain/1
  Complex to Real-Imag/1 -> Product2/2
  Product2/1 -> Sum1/1
  Sum1/1 -> ref/1  "i"
  Gain/1 -> Complex to Real-Imag/1
  Complex to Real-Imag/2 -> Product1/2
  Product1/1 -> Sum1/2
  cmd/1 -> Complex to Real-Imag1/1
  Complex to Real-Imag1/1 -> Product2/1
  Complex to Real-Imag1/2 -> Product1/1

== system My_gfm_battery_sil_2_ConvIGBT_zDomain/My Inverter Controller /My_machineModel_A1/governer/LPF(DamperDecoupler) limited  ==
  In : Inport
  1/tau_damp : Gain  Gain=1/0.3
  Integrator : Integrator  LimitOutput=on  UpperSaturationLimit=1.2*SRated  LowerSaturationLimit=-1.2*SRated
  Sum3 : Sum  Inputs=|+-
  Out : Outport
  wires:
  Integrator/1 -> Out/1, Sum3/2
  Sum3/1 -> 1/tau_damp/1
  In/1 -> Sum3/1
  1/tau_damp/1 -> Integrator/1

== system My_gfm_battery_sil_2_ConvIGBT_zDomain/My Inverter Controller /My_machineModel_A1/governer/synchronizer ==
  note: Why?
  note: Big Range?
  note: prevent it from acting during typical faults
  note: Prevent loss of sync at low voltage events, using asym filter to traget long extended low voltage events
  note: Keeps the machine spining in synchronize while machine is disabled, disabling the machine means
  note: Why?
  Vq : Inport
  Vt : Inport  Port=2
  machine_enabled : Inport  Port=3
  Constant : Constant
  Gain : Gain  Gain=SRated
  Gain2 : Gain  Gain=1/VllRated
  HPF : Subsystem
  Product1 : Product
  Saturation : Saturate  UpperLimit=1  LowerLimit=0
  Sum : Sum  Inputs=|++
  Sum2 : Sum  Inputs=|+-
  Switch : Switch  Criteria=u2 > Threshold  SaturateOnIntegerOverflow=off  InputSameDT=off
  Transfer Fcn : TransferFcn  Commented=on  Numerator=[(2 * pi * 50) 0]  Denominator=[1, (2*pi*50)]
  assymmetric filter1 : Subsystem
  gain : Gain  Gain=2*pi*50
  kFastSync : Gain
  kSync : Gain  Gain=20
  pSyncLimit : Saturate  UpperLimit=3  LowerLimit=-3
  syncFadeGain : Gain  Gain=4
  syncFadeThreshold : Constant  Value=0.2
  to_pu : Gain  Gain=1 / VllRated
  p_sync_pu : Outport
  wires:
  to_pu/1 -> Sum2/2
  Vt/1 -> assymmetric filter1/1(in)
  assymmetric filter1/1(out) -> to_pu/1
  pSyncLimit/1 -> Gain/1
  kSync/1 -> Sum/1
  Sum/1 -> pSyncLimit/1
  Product1/1 -> p_sync_pu/1
  Constant/1 -> Switch/3
  Sum2/1 -> syncFadeGain/1
  machine_enabled/1 -> Switch/2
  syncFadeGain/1 -> Saturation/1
  Saturation/1 -> Switch/1
  syncFadeThreshold/1 -> Sum2/1
  Switch/1 -> Product1/2
  Gain2/1 -> kFastSync/1, kSync/1
  Vq/1 -> Gain2/1
  Gain/1 -> Product1/1  "p_sync"
  kFastSync/1 -> HPF/1(in)
  HPF/1(out) -> gain/1
  gain/1 -> Sum/2

== system My_gfm_battery_sil_2_ConvIGBT_zDomain/My Inverter Controller /My_machineModel_A1/governer1/LPF(DamperDecoupler) - limited ==
  In1 : Inport
  Integrator : Integrator  LimitOutput=on  UpperSaturationLimit=1.2*SRated  LowerSaturationLimit=-1.2*SRated
  Sum3 : Sum  Inputs=|+-
  wDamperDecoupler : Gain  Gain=1/0.3
  Out1 : Outport
  wires:
  Integrator/1 -> Out1/1, Sum3/2
  Sum3/1 -> wDamperDecoupler/1
  wDamperDecoupler/1 -> Integrator/1
  In1/1 -> Sum3/1

== system My_gfm_battery_sil_2_ConvIGBT_zDomain/My Inverter Controller /My_machineModel_A1/governer1/LPF(DamperDecoupler) limited 1 ==
  In : Inport
  1/tau_damp : Gain  Gain=1/0.3
  Integrator : Integrator  LimitOutput=on  UpperSaturationLimit=1.2*SRated  LowerSaturationLimit=-1.2*SRated
  Sum3 : Sum  Inputs=|+-
  Out : Outport
  wires:
  Integrator/1 -> Out/1, Sum3/2
  Sum3/1 -> 1/tau_damp/1
  In/1 -> Sum3/1
  1/tau_damp/1 -> Integrator/1

== system My_gfm_battery_sil_2_ConvIGBT_zDomain/My Inverter Controller /My_machineModel_A1/governer1/synchronizer ==
  note: Why?
  note: Big Range?
  note: prevent it from acting during typical faults
  note: Prevent loss of sync at low voltage events, using asym filter to traget long extended low voltage events
  note: Keeps the machine spining in synchronize while machine is disabled, disabling the machine means
  note: Why?
  note: Should be sqrt(Vd^2 + Vq^2) ?
  Vq : Inport
  Vd : Inport  Port=2
  machine_enabled : Inport  Port=3
  Constant : Constant
  Gain : Gain  Gain=SRated
  Gain2 : Gain  Gain=1/VllRated
  HPF : Subsystem
  Product1 : Product
  Saturation : Saturate  UpperLimit=1  LowerLimit=0
  Sum : Sum  Inputs=|++
  Sum2 : Sum  Inputs=|+-
  Switch : Switch  Criteria=u2 > Threshold  SaturateOnIntegerOverflow=off  InputSameDT=off
  Transfer Fcn : TransferFcn  Commented=on  Numerator=[(2 * pi * 50) 0]  Denominator=[1, (2*pi*50)]
  assymmetric filter1 : Subsystem
  gain : Gain  Gain=2*pi*50
  kFastSync : Gain
  kSync : Gain  Gain=20
  pSyncLimit : Saturate  UpperLimit=3  LowerLimit=-3
  syncFadeGain : Gain  Gain=4
  syncFadeThreshold : Constant  Value=0.2
  to_pu : Gain  Gain=1 / VllRated
  p_sync_pu : Outport
  wires:
  to_pu/1 -> Sum2/2
  Vd/1 -> assymmetric filter1/1(in)
  assymmetric filter1/1(out) -> to_pu/1
  pSyncLimit/1 -> Gain/1
  kSync/1 -> Sum/1
  Sum/1 -> pSyncLimit/1
  Product1/1 -> p_sync_pu/1
  Constant/1 -> Switch/3
  Sum2/1 -> syncFadeGain/1
  machine_enabled/1 -> Switch/2
  syncFadeGain/1 -> Saturation/1
  Saturation/1 -> Switch/1
  syncFadeThreshold/1 -> Sum2/1
  Switch/1 -> Product1/2
  Gain2/1 -> kFastSync/1, kSync/1
  Vq/1 -> Gain2/1
  Gain/1 -> Product1/1  "p_sync"
  kFastSync/1 -> HPF/1(in)
  HPF/1(out) -> gain/1
  gain/1 -> Sum/2

== system My_gfm_battery_sil_2_ConvIGBT_zDomain/My Inverter Controller /My_machineModel_A1/rotor model/HPF (wDamperDecoupler) 1 ==
  in : Inport
  1/tau_damp : Gain  Gain=1/0.3
  Integrator : Integrator
  Sum : Sum  Inputs=|+-
  out : Outport
  wires:
  Sum/1 -> out/1, 1/tau_damp/1
  in/1 -> Sum/1
  Integrator/1 -> Sum/2
  1/tau_damp/1 -> Integrator/1

== system My_gfm_battery_sil_2_ConvIGBT_zDomain/My Inverter Controller /My_machineModel_A1/rotor model/oscillator_3ph ==
  f : Inport
  Cos : Trigonometry  Operator=cos
  Gain : Gain  Gain=2*pi
  Integrator : Integrator
  Real-Imag to Complex : RealImagToComplex
  Sin : Trigonometry
  Sum1 : Sum  Inputs=|++
  phase_shift : Constant  Value=[0 -1/3 -2/3]
  osc[3] : Outport
  wires:
  f/1 -> Integrator/1
  Real-Imag to Complex/1 -> osc[3]/1
  Cos/1 -> Real-Imag to Complex/1
  Gain/1 -> Cos/1, Sin/1
  Integrator/1 -> Sum1/1
  Sin/1 -> Real-Imag to Complex/2
  phase_shift/1 -> Sum1/2
  Sum1/1 -> Gain/1

== system My_gfm_battery_sil_2_ConvIGBT_zDomain/Plant controller (simplified example)/Meter/PLL-analog/oscillator_3ph ==
  f : Inport
  Cos : Trigonometry  Operator=cos
  Gain : Gain  Gain=2*pi
  Integrator : Integrator
  Real-Imag to Complex : RealImagToComplex
  Sin : Trigonometry
  Sum1 : Sum  Inputs=|++
  phase_shift : Constant  Value=[0 -1/3 -2/3]
  osc[3] : Outport
  wires:
  Sum1/1 -> Gain/1
  phase_shift/1 -> Sum1/2
  Sin/1 -> Real-Imag to Complex/2
  Integrator/1 -> Sum1/1
  Gain/1 -> Sin/1, Cos/1
  Cos/1 -> Real-Imag to Complex/1
  Real-Imag to Complex/1 -> osc[3]/1
  f/1 -> Integrator/1

== system My_gfm_battery_sil_2_ConvIGBT_zDomain/ac Network with MVT (native math)4/powergui/EquivalentModel1/Sources ==
  Mux : Mux  Inputs=[1 1 1 1 1 1]
  u : Outport  VectorParamsAs1DForOutWhenUnconnected=off
  wires:
  Mux/1 -> u/1
  [T110_10072_18540693045835] -> Mux/1
  [T110_10073_18546958997832] -> Mux/2
  [T110_10074_18553562230555] -> Mux/3
  [T104_9471_15257157992367] -> Mux/4
  [T104_9472_15263231413055] -> Mux/5
  [T105_9521_15201317903447] -> Mux/6

== system My_gfm_battery_sil_2_ConvIGBT_zDomain/ac Network with MVT (native math)4/powergui/EquivalentModel1/Yout ==
  v,i : Inport
  Demux : Demux  Outputs=[1 1 1 1 1 1 1 1 1 1 1 1 1 1 1 1 1]
  tag scope: T101_8788_13506312305887=global, T101_8789_13512331616667=global, T101_8790_13518638934576=global, T101_8800_13617096052105=global, T101_8801_13623081547123=global, T101_8802_13629355049269=global, T102_8863_13653826365305=global, T102_8864_13659950384888=global, T102_8865_13666365769374=global, T102_8875_13766394121088=global, T102_8876_13772484261417=global, T102_8877_13778865766648=global, T114_10480_19873251167167=global, T114_10482_19885120530449=global, T127_11890_28685161815829=global, T128_11939_28594174590354=global, T128_11940_28594194970608=global
  wires:
  v,i/1 -> Demux/1
  Demux/1 -> [T102_8875_13766394121088]
  Demux/2 -> [T102_8876_13772484261417]
  Demux/3 -> [T102_8877_13778865766648]
  Demux/4 -> [T101_8800_13617096052105]
  Demux/5 -> [T101_8801_13623081547123]
  Demux/6 -> [T101_8802_13629355049269]
  Demux/7 -> [T114_10480_19873251167167]
  Demux/8 -> [T114_10482_19885120530449]
  Demux/9 -> [T102_8863_13653826365305]
  Demux/10 -> [T102_8864_13659950384888]
  Demux/11 -> [T102_8865_13666365769374]
  Demux/12 -> [T101_8788_13506312305887]
  Demux/13 -> [T101_8789_13512331616667]
  Demux/14 -> [T101_8790_13518638934576]
  Demux/15 -> [T127_11890_28685161815829]
  Demux/16 -> [T128_11939_28594174590354]
  Demux/17 -> [T128_11940_28594194970608]

== system My_gfm_battery_sil_2_ConvIGBT_zDomain/ac Network with MVT (native math)4/powergui/EquivalentModel2/Sources ==
  Mux : Mux  Inputs=[1 1 1 1 1 1]
  u : Outport  VectorParamsAs1DForOutWhenUnconnected=off
  wires:
  Mux/1 -> u/1
  [T127_11776_26356052463873] -> Mux/1
  [T128_11825_26229814574488] -> Mux/2
  [T85_7683_9614987755625] -> Mux/3
  [T85_7684_9619946320720] -> Mux/4
  [T85_7685_9615963782852] -> Mux/5
  [T85_7686_9620916550042] -> Mux/6

== system My_gfm_battery_sil_2_ConvIGBT_zDomain/ac Network with MVT (native math)4/powergui/EquivalentModel2/Yout ==
  v,i : Inport
  Demux : Demux  Outputs=[1 1 1 1 1 1 1 1 1 1 1 1 1 1 1 1 1 1]
  tag scope: T101_8844_13845888351347=global, T101_8845_13851766681921=global, T101_8846_13857933019624=global, T101_8856_13955016807584=global, T101_8857_13960861322396=global, T101_8858_13966993844337=global, T102_8884_13951931031537=global, T102_8885_13957994439534=global, T102_8886_13964349212434=global, T102_8896_14063786961671=global, T102_8897_14069816490414=global, T102_8898_14076137384058=global, T127_11925_28478252064881=global, T128_11974_28388591653140=global, T128_11975_28388555561297=global, T94_8644_13498791624137=global, T94_8646_13507986467916=global, T95_8695_13502152486009=global
  wires:
  v,i/1 -> Demux/1
  Demux/1 -> [T102_8896_14063786961671]
  Demux/2 -> [T102_8897_14069816490414]
  Demux/3 -> [T102_8898_14076137384058]
  Demux/4 -> [T101_8856_13955016807584]
  Demux/5 -> [T101_8857_13960861322396]
  Demux/6 -> [T101_8858_13966993844337]
  Demux/7 -> [T94_8644_13498791624137]
  Demux/8 -> [T94_8646_13507986467916]
  Demux/9 -> [T95_8695_13502152486009]
  Demux/10 -> [T102_8884_13951931031537]
  Demux/11 -> [T102_8885_13957994439534]
  Demux/12 -> [T102_8886_13964349212434]
  Demux/13 -> [T101_8844_13845888351347]
  Demux/14 -> [T101_8845_13851766681921]
  Demux/15 -> [T101_8846_13857933019624]
  Demux/16 -> [T127_11925_28478252064881]
  Demux/17 -> [T128_11974_28388591653140]
  Demux/18 -> [T128_11975_28388555561297]

== system My_gfm_battery_sil_2_ConvIGBT_zDomain/ac Network with MVT (native math)4/powergui/EquivalentModel3/Sources ==
  Mux : Mux  Inputs=[1 1]
  u : Outport  VectorParamsAs1DForOutWhenUnconnected=off
  wires:
  Mux/1 -> u/1
  [T103_9651_17767016193933] -> Mux/1
  [T108_9898_18128775488598] -> Mux/2

== system My_gfm_battery_sil_2_ConvIGBT_zDomain/ac Network with MVT (native math)4/powergui/EquivalentModel3/Yout ==
  v,i : Inport
  Demux : Demux  Outputs=[1 1]
  tag scope: T112_10295_19938657508366=global, T99_9354_17225524064677=global
  wires:
  v,i/1 -> Demux/1
  Demux/1 -> [T112_10295_19938657508366]
  Demux/2 -> [T99_9354_17225524064677]

== system My_gfm_battery_sil_2_ConvIGBT_zDomain/My Inverter Controller /My_machineModel_A/governer/synchronizer/HPF  ==
  in : Inport
  Integrator : Integrator
  Sum : Sum  Inputs=|+-
  wSync : Gain  Gain=wSync
  out : Outport
  wires:
  Sum/1 -> out/1, wSync/1
  in/1 -> Sum/1
  Integrator/1 -> Sum/2
  wSync/1 -> Integrator/1

== system My_gfm_battery_sil_2_ConvIGBT_zDomain/My Inverter Controller /My_machineModel_A/governer/synchronizer/assymmetric filter1 ==
  note: The saturation block is configured to cause a rapid rise, but much slow drop in output.
  in : Inport
  Gain1 : Gain  Gain=1/tauBkSt
  Integrator : Integrator
  Saturation1 : Saturate  UpperLimit=VllRated  LowerLimit=-0.02 * VllRated
  Sum3 : Sum  Inputs=|+-
  out : Outport
  wires:
  Integrator/1 -> out/1, Sum3/2
  Sum3/1 -> Gain1/1
  in/1 -> Sum3/1
  Gain1/1 -> Saturation1/1
  Saturation1/1 -> Integrator/1

== system My_gfm_battery_sil_2_ConvIGBT_zDomain/My Inverter Controller /My_machineModel_A1/governer/synchronizer/HPF ==
  in : Inport
  1/tau : Gain  Gain=2*pi*50
  Integrator : Integrator
  Sum : Sum  Inputs=|+-
  out : Outport
  wires:
  Sum/1 -> out/1, 1/tau/1
  in/1 -> Sum/1
  Integrator/1 -> Sum/2
  1/tau/1 -> Integrator/1

== system My_gfm_battery_sil_2_ConvIGBT_zDomain/My Inverter Controller /My_machineModel_A1/governer/synchronizer/assymmetric filter1 ==
  note: The saturation block is configured to cause a rapid rise, but much slow drop in output.
  in : Inport
  Gain1 : Gain  Gain=2
  Integrator : Integrator
  Saturation1 : Saturate  UpperLimit=VllRated  LowerLimit=-0.02 * VllRated
  Sum3 : Sum  Inputs=|+-
  out : Outport
  wires:
  Integrator/1 -> out/1, Sum3/2
  Sum3/1 -> Gain1/1
  in/1 -> Sum3/1
  Gain1/1 -> Saturation1/1
  Saturation1/1 -> Integrator/1

== system My_gfm_battery_sil_2_ConvIGBT_zDomain/My Inverter Controller /My_machineModel_A1/governer1/synchronizer/HPF ==
  in : Inport
  1/tau : Gain  Gain=2*pi*50
  Integrator : Integrator
  Sum : Sum  Inputs=|+-
  out : Outport
  wires:
  Sum/1 -> out/1, 1/tau/1
  in/1 -> Sum/1
  Integrator/1 -> Sum/2
  1/tau/1 -> Integrator/1

== system My_gfm_battery_sil_2_ConvIGBT_zDomain/My Inverter Controller /My_machineModel_A1/governer1/synchronizer/assymmetric filter1 ==
  note: The saturation block is configured to cause a rapid rise, but much slow drop in output.
  in : Inport
  Gain1 : Gain  Gain=2
  Integrator : Integrator
  Saturation1 : Saturate  UpperLimit=VllRated  LowerLimit=-0.02 * VllRated
  Sum3 : Sum  Inputs=|+-
  out : Outport
  wires:
  Integrator/1 -> out/1, Sum3/2
  Sum3/1 -> Gain1/1
  in/1 -> Sum3/1
  Gain1/1 -> Saturation1/1
  Saturation1/1 -> Integrator/1

== matlab function My_gfm_battery_sil_2_ConvIGBT_zDomain/ac Network with MVT (native math)4/Two-Level Converter1/Model1/MATLAB Function ==
  data: g input; V output; Vdc input; I input; Idc output
function [V,Idc] = FunctionHalfBridge1(g,Vdc,I)
[V,Idc]=FunctionHalfBridge(g,Vdc,I);

== matlab function My_gfm_battery_sil_2_ConvIGBT_zDomain/ac Network with MVT (native math)4/Two-Level Converter1/Model2/MATLAB Function ==
  data: g input; V output; Vdc input; I input; Idc output
function [V,Idc] = FunctionHalfBridge1(g,Vdc,I)
[V,Idc]=FunctionHalfBridge(g,Vdc,I);

== matlab function My_gfm_battery_sil_2_ConvIGBT_zDomain/ac Network with MVT (native math)4/Two-Level Converter1/Model3/MATLAB Function ==
  data: g input; V output; Vdc input; I input; Idc output
function [V,Idc] = FunctionHalfBridge1(g,Vdc,I)
[V,Idc]=FunctionHalfBridge(g,Vdc,I);

== matlab function My_gfm_battery_sil_2_ConvIGBT_zDomain/ac Network with MVT (native math)3/Two-Level Converter/Model1/MATLAB Function ==
  data: g input; V output; Vdc input; I input; Idc output
function [V,Idc] = FunctionHalfBridge1(g,Vdc,I)
[V,Idc]=FunctionHalfBridge(g,Vdc,I);

== matlab function My_gfm_battery_sil_2_ConvIGBT_zDomain/ac Network with MVT (native math)3/Two-Level Converter/Model2/MATLAB Function ==
  data: g input; V output; Vdc input; I input; Idc output
function [V,Idc] = FunctionHalfBridge1(g,Vdc,I)
[V,Idc]=FunctionHalfBridge(g,Vdc,I);

== matlab function My_gfm_battery_sil_2_ConvIGBT_zDomain/ac Network with MVT (native math)3/Two-Level Converter/Model3/MATLAB Function ==
  data: g input; V output; Vdc input; I input; Idc output
function [V,Idc] = FunctionHalfBridge1(g,Vdc,I)
[V,Idc]=FunctionHalfBridge(g,Vdc,I);
